simulink model "Closed_Loop"  (R2024b)
settings: Solver=VariableStepAuto  StartTime=0.0  StopTime=10  MaxStep=0.01  RelTol=1e-3
settings Model: LastModifiedBy=devan
settings ModelReferenceCC: UpdateModelReferenceTargets=IfOutOfDate

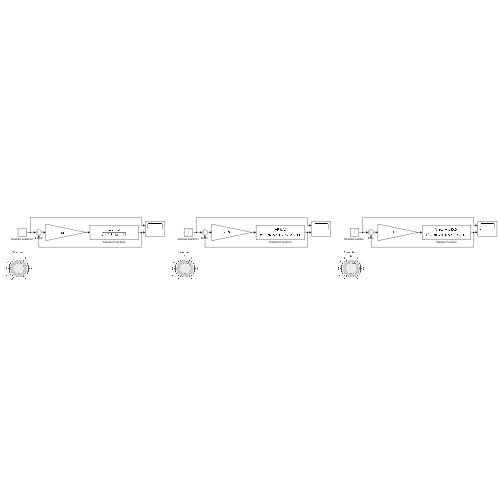
[thumbnail: Simulink's stored preview of the top-level diagram]
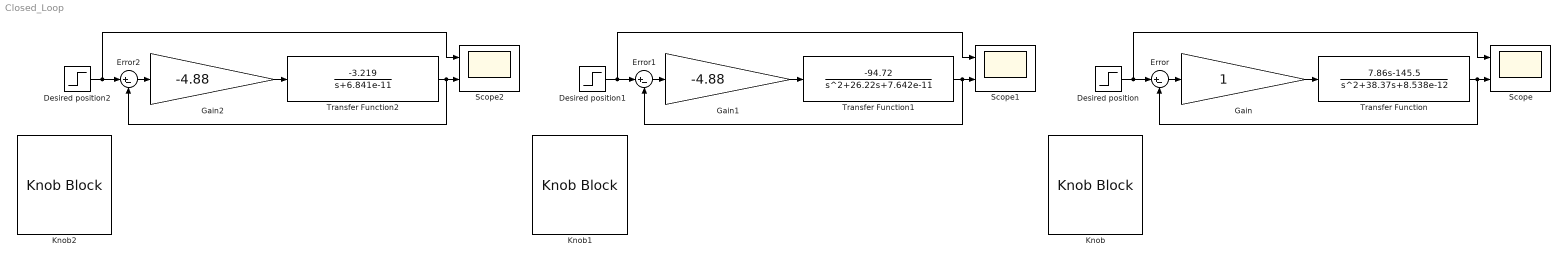
== system Closed_Loop ==
  Desired position : Step  Time=0  SampleTime=0
  Desired position1 : Step  Time=0  SampleTime=0
  Desired position2 : Step  Time=0  SampleTime=0
  Error : Sum  Inputs=|+-
  Error1 : Sum  Inputs=|+-
  Error2 : Sum  Inputs=|+-
  Gain : Gain
  Gain1 : Gain  Gain=-4.88
  Gain2 : Gain  Gain=-4.88
  Knob : KnobBlock  ScaleMin=-5  ScaleMax=5
  Knob1 : KnobBlock  ScaleMin=-5  ScaleMax=5
  Knob2 : KnobBlock  ScaleMin=-5  ScaleMax=5
  Scope : Scope  NumInputPorts=2
  Scope1 : Scope  NumInputPorts=2
  Scope2 : Scope  NumInputPorts=2
  Transfer Function : TransferFcn  Numerator=[7.86 -145.5]  Denominator=[1 38.37 8.538e-12]
  Transfer Function1 : TransferFcn  Numerator=[-94.72]  Denominator=[1 26.22 7.642e-11]
  Transfer Function2 : TransferFcn  Numerator=[-3.219]  Denominator=[1 6.841e-11]
  wires:
  Desired position/1 -> Error/1, Scope/1
  Error/1 -> Gain/1
  Gain/1 -> Transfer Function/1
  Transfer Function/1 -> Error/2, Scope/2
  Gain1/1 -> Transfer Function1/1
  Desired position1/1 -> Error1/1, Scope1/1
  Error1/1 -> Gain1/1
  Transfer Function1/1 -> Error1/2, Scope1/2
  Error2/1 -> Gain2/1
  Transfer Function2/1 -> Error2/2, Scope2/2
  Gain2/1 -> Transfer Function2/1
  Desired position2/1 -> Error2/1, Scope2/1
